simulink model "DemoPromo"  (R2025b)
settings: Solver=VariableStepAuto  StartTime=0.0  StopTime=10.0  RelTol=1e-3
settings Model: Creator=Edward  LastModifiedBy=Edward

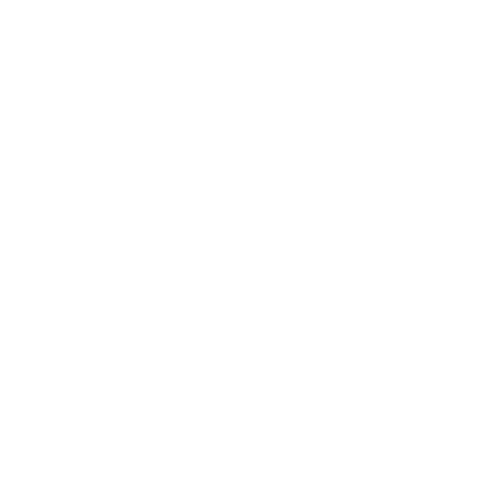
[thumbnail: Simulink's stored preview of the top-level diagram]
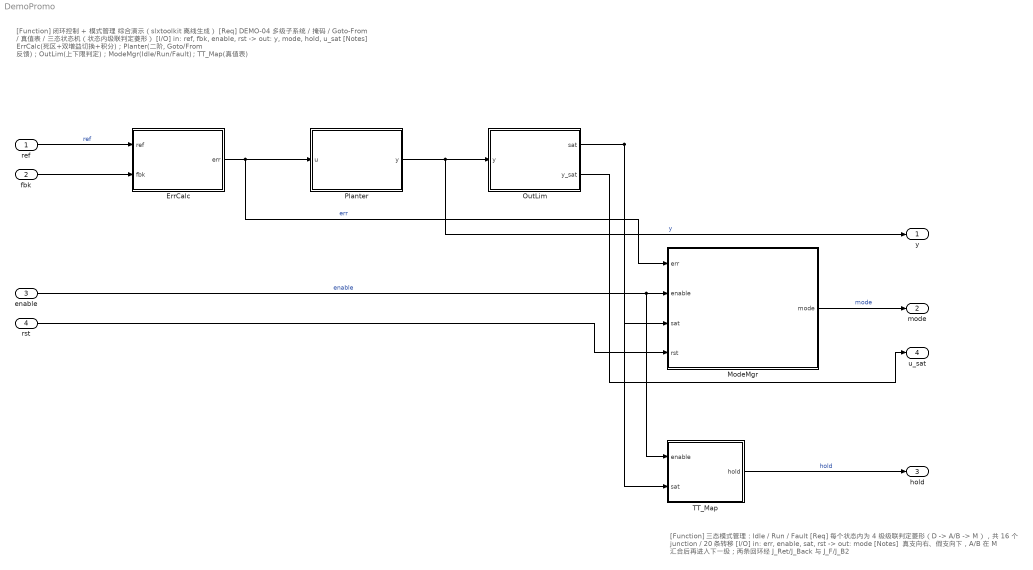
== system DemoPromo ==
  note: [Function] 闭环控制 + 模式管理 综合演示（slxtoolkit 离线生成）
      | [Req] DEMO-04 多级子系统 / 掩码 / Goto-From / 真值表 / 三态状态机（状态内级联判定菱形）
      | [I/O] in: ref, fbk, enable, rst -> out: y, mode, hold, u_sat
      | [Notes] ErrCalc(死区+双增益切换+积分)；Planter(二阶, Goto/From 反馈)；OutLim(上下限判定)；ModeMgr(Idle/Run/Fault)；TT_Map(真值表)
  note: [Function] 三态模式管理：Idle / Run / Fault
      | [Req] 每个状态内为 4 级级联判定菱形（D -> A/B -> M），共 16 个 junction / 20 条转移
      | [I/O] in: err, enable, sat, rst -> out: mode
      | [Notes] 真支向右、假支向下，A/B 在 M 汇合后再进入下一级；两条回环经 J_Ret/J_Back 与 J_F/J_B2
  ref : Inport  OutDataTypeStr=single  PortDimensions=1
  fbk : Inport  OutDataTypeStr=single  PortDimensions=1  Port=2
  enable : Inport  OutDataTypeStr=boolean  PortDimensions=1  Port=3
  rst : Inport  OutDataTypeStr=boolean  PortDimensions=1  Port=4
  ErrCalc : Subsystem  mask(PI Error Calc){Kp=1.5, Kp2=3.0, Ki=0.25}
      mask prompts: Kp "比例增益 Kp"; Kp2 "大误差增益 Kp2"; Ki "积分增益 Ki"
      mask help: 比例 / 积分误差计算（含死区与大误差增益切换），Kp / Kp2 / Ki 由掩码参数给定
      mask DialogControl G_Gain Prompt: PI 增益
      mask DialogControl T_Info Prompt: 仅标定用，运行期不可调
      mask Display: disp('PI error: deadband -> Kp/Kp2 boost -> + Ki integral')
  ModeMgr : Stateflow chart  TreatAsAtomicUnit=on
  OutLim : Subsystem
  Planter : Subsystem
  TT_Map : Truth Table  TreatAsAtomicUnit=on
  y : Outport  OutDataTypeStr=single  PortDimensions=1
  mode : Outport  OutDataTypeStr=uint8  PortDimensions=1  Port=2
  hold : Outport  OutDataTypeStr=boolean  PortDimensions=1  Port=3
  u_sat : Outport  OutDataTypeStr=single  PortDimensions=1  Port=4
  wires:
  ref/1 -> ErrCalc/1(ref)  "ref"
  fbk/1 -> ErrCalc/2(fbk)
  ErrCalc/1(err) -> Planter/1(u), ModeMgr/1(err)  "err"
  Planter/1(y) -> OutLim/1(y), y/1  "y"
  OutLim/1(sat) -> ModeMgr/3(sat), TT_Map/2(sat)
  OutLim/2(y_sat) -> u_sat/1
  enable/1 -> ModeMgr/2(enable), TT_Map/1(enable)  "enable"
  rst/1 -> ModeMgr/4(rst)
  ModeMgr/1(mode) -> mode/1  "mode"
  TT_Map/1(hold) -> hold/1  "hold"

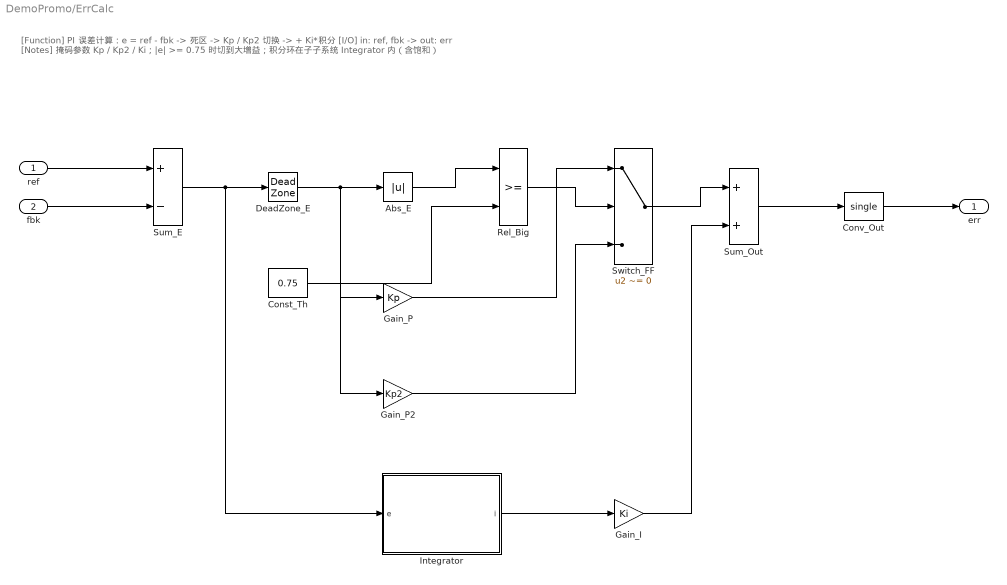
== system DemoPromo/ErrCalc ==
  note: [Function] PI 误差计算：e = ref - fbk -> 死区 -> Kp / Kp2 切换 -> + Ki*积分
      | [I/O] in: ref, fbk -> out: err
      | [Notes] 掩码参数 Kp / Kp2 / Ki；|e| >= 0.75 时切到大增益；积分环在子子系统 Integrator 内（含饱和）
  ref : Inport  OutDataTypeStr=single  PortDimensions=1
  fbk : Inport  OutDataTypeStr=single  PortDimensions=1  Port=2
  Abs_E : Abs
  Const_Th : Constant  Value=0.75  OutDataTypeStr=single  SampleTime=-1
  Conv_Out : DataTypeConversion  OutDataTypeStr=single
  DeadZone_E : DeadZone  LowerValue=-0.0625  UpperValue=0.0625
  Gain_I : Gain  Gain=Ki  OutDataTypeStr=single
  Gain_P : Gain  Gain=Kp  OutDataTypeStr=single
  Gain_P2 : Gain  Gain=Kp2  OutDataTypeStr=single
  Integrator : Subsystem
  Rel_Big : RelationalOperator
  Sum_E : Sum  Inputs=+-
  Sum_Out : Sum
  Switch_FF : Switch  Criteria=u2 ~= 0
  err : Outport  OutDataTypeStr=single  PortDimensions=1
  wires:
  ref/1 -> Sum_E/1
  fbk/1 -> Sum_E/2
  Sum_E/1 -> DeadZone_E/1, Integrator/1(e)
  DeadZone_E/1 -> Abs_E/1, Gain_P/1, Gain_P2/1
  Abs_E/1 -> Rel_Big/1
  Const_Th/1 -> Rel_Big/2
  Gain_P/1 -> Switch_FF/1
  Rel_Big/1 -> Switch_FF/2
  Gain_P2/1 -> Switch_FF/3
  Switch_FF/1 -> Sum_Out/1
  Integrator/1(i) -> Gain_I/1
  Gain_I/1 -> Sum_Out/2
  Sum_Out/1 -> Conv_Out/1
  Conv_Out/1 -> err/1

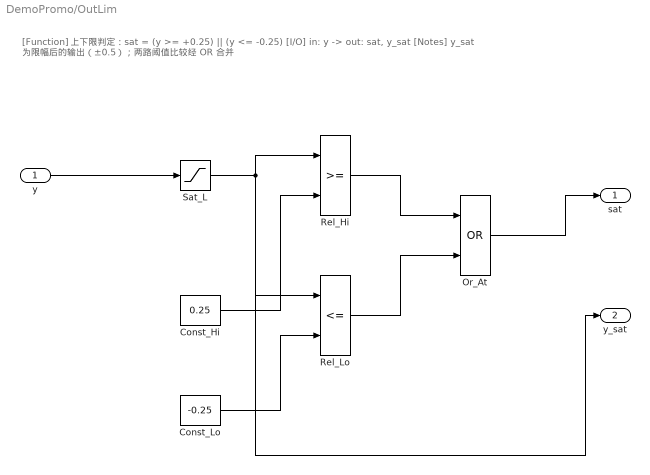
== system DemoPromo/OutLim ==
  note: [Function] 上下限判定：sat = (y >= +0.25) || (y <= -0.25)
      | [I/O] in: y -> out: sat, y_sat
      | [Notes] y_sat 为限幅后的输出（±0.5）；两路阈值比较经 OR 合并
  y : Inport  OutDataTypeStr=single  PortDimensions=1
  Const_Hi : Constant  Value=0.25  OutDataTypeStr=single  SampleTime=-1
  Const_Lo : Constant  Value=-0.25  OutDataTypeStr=single  SampleTime=-1
  Or_At : Logic  Operator=OR
  Rel_Hi : RelationalOperator
  Rel_Lo : RelationalOperator  Operator=<=
  Sat_L : Saturate
  sat : Outport  OutDataTypeStr=boolean  PortDimensions=1
  y_sat : Outport  OutDataTypeStr=single  PortDimensions=1  Port=2
  wires:
  y/1 -> Sat_L/1
  Sat_L/1 -> Rel_Hi/1, Rel_Lo/1, y_sat/1
  Const_Hi/1 -> Rel_Hi/2
  Const_Lo/1 -> Rel_Lo/2
  Rel_Hi/1 -> Or_At/1
  Rel_Lo/1 -> Or_At/2
  Or_At/1 -> sat/1

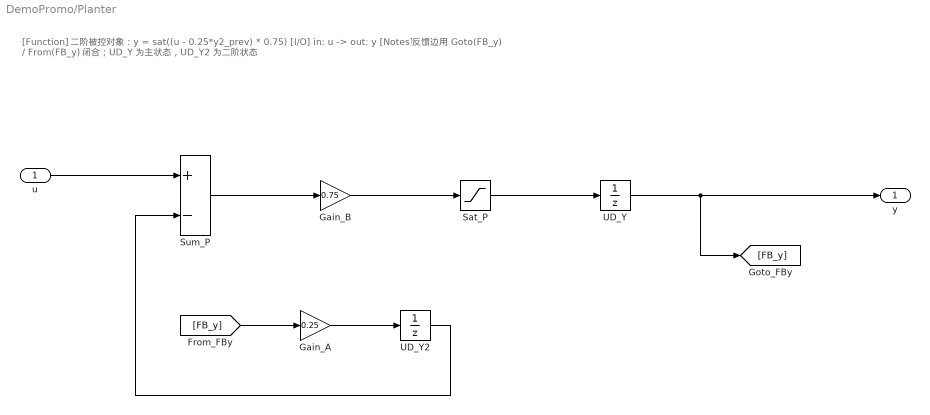
== system DemoPromo/Planter ==
  note: [Function] 二阶被控对象：y = sat((u - 0.25*y2_prev) * 0.75)
      | [I/O] in: u -> out: y
      | [Notes] 反馈边用 Goto(FB_y) / From(FB_y) 闭合；UD_Y 为主状态，UD_Y2 为二阶状态
  u : Inport  OutDataTypeStr=single  PortDimensions=1
  Gain_A : Gain  Gain=0.25  OutDataTypeStr=single
  Gain_B : Gain  Gain=0.75  OutDataTypeStr=single
  Sat_P : Saturate  UpperLimit=1.0  LowerLimit=-1.0
  Sum_P : Sum  Inputs=+-
  UD_Y : UnitDelay  SampleTime=-1
  UD_Y2 : UnitDelay  SampleTime=-1
  y : Outport  OutDataTypeStr=single  PortDimensions=1
  wires:
  u/1 -> Sum_P/1
  Sum_P/1 -> Gain_B/1
  Gain_B/1 -> Sat_P/1
  Sat_P/1 -> UD_Y/1
  UD_Y/1 -> y/1, [FB_y]
  [FB_y] -> Gain_A/1
  Gain_A/1 -> UD_Y2/1
  UD_Y2/1 -> Sum_P/2

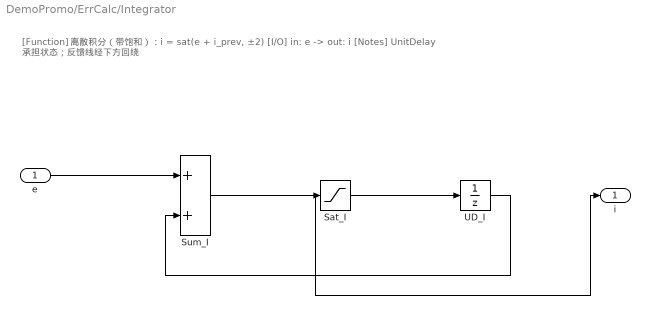
== system DemoPromo/ErrCalc/Integrator ==
  note: [Function] 离散积分（带饱和）：i = sat(e + i_prev, ±2)
      | [I/O] in: e -> out: i
      | [Notes] UnitDelay 承担状态；反馈线经下方回绕
  e : Inport  OutDataTypeStr=single  PortDimensions=1
  Sat_I : Saturate  UpperLimit=2.0  LowerLimit=-2.0
  Sum_I : Sum
  UD_I : UnitDelay  SampleTime=-1
  i : Outport  OutDataTypeStr=single  PortDimensions=1
  wires:
  e/1 -> Sum_I/1
  Sum_I/1 -> Sat_I/1, i/1
  Sat_I/1 -> UD_I/1
  UD_I/1 -> Sum_I/2

== stateflow chart DemoPromo/ModeMgr ==
  state Idle
    en: mode = uint8(0);
    (default) -> (junction 22)
    (junction 22) -> (junction 23) [order 1] : [err < 0.10]
    (junction 22) -> (junction 24) [order 2]
    (junction 23) -> (junction 25)
    (junction 24) -> (junction 25)
    (junction 25) -> (junction 26)
    (junction 26) -> (junction 27) [order 1] : [err < 0.20]
    (junction 26) -> (junction 28) [order 2]
    (junction 27) -> (junction 29)
    (junction 28) -> (junction 29)
    (junction 29) -> (junction 30)
    (junction 30) -> (junction 31) [order 1] : [err < 0.35]
    (junction 30) -> (junction 32) [order 2]
    (junction 31) -> (junction 33)
    (junction 32) -> (junction 33)
    (junction 33) -> (junction 34)
    (junction 34) -> (junction 35) [order 1] : [err < 0.50]
    (junction 34) -> (junction 36) [order 2]
    (junction 35) -> (junction 37)
    (junction 36) -> (junction 37)
  state Run
    en: mode = uint8(1);
    (default) -> (junction 58)
    (junction 58) -> (junction 59) [order 1] : [err < 0.60]
    (junction 58) -> (junction 60) [order 2]
    (junction 59) -> (junction 61)
    (junction 60) -> (junction 61)
    (junction 61) -> (junction 62)
    (junction 62) -> (junction 63) [order 1] : [err < 0.70]
    (junction 62) -> (junction 64) [order 2]
    (junction 63) -> (junction 65)
    (junction 64) -> (junction 65)
    (junction 65) -> (junction 66)
    (junction 66) -> (junction 67) [order 1] : [err < 0.80]
    (junction 66) -> (junction 68) [order 2]
    (junction 67) -> (junction 69)
    (junction 68) -> (junction 69)
    (junction 69) -> (junction 70)
    (junction 70) -> (junction 71) [order 1] : [err < 0.90]
    (junction 70) -> (junction 72) [order 2]
    (junction 71) -> (junction 73)
    (junction 72) -> (junction 73)
  state Fault
    en: mode = uint8(2);
    (default) -> (junction 94)
    (junction 94) -> (junction 95) [order 1] : [err < 0]
    (junction 94) -> (junction 96) [order 2]
    (junction 95) -> (junction 97)
    (junction 96) -> (junction 97)
  (default) -> Idle
  Idle -> Run : [enable]
  Run -> Fault [order 2] : [sat]
  Fault -> (junction 11) : [rst]{mode = uint8(0);}
  (junction 10) -> Idle
  Run -> (junction 9) [order 1] : [enable == false]
  (junction 9) -> (junction 10)
  (junction 12) -> (junction 10)
  (junction 11) -> (junction 12)
  data: err input single size=1; enable input boolean size=1; sat input boolean size=1; rst input boolean size=1; mode output uint8 size=1

== matlab function DemoPromo/TT_Map ==
  data: enable input boolean; sat input boolean; hold output boolean
function hold = fcn(enable, sat)

aVarTruthTableCondition_1 = false;
aVarTruthTableCondition_2 = false;


% 使能

aVarTruthTableCondition_1 = logical(enable);

% 饱和

aVarTruthTableCondition_2 = logical(sat);

if (aVarTruthTableCondition_1 && aVarTruthTableCondition_2)
    aFcnTruthTableAction_1();
elseif (aVarTruthTableCondition_1 && ~aVarTruthTableCondition_2)
    aFcnTruthTableAction_2();
else % Default
    aFcnTruthTableAction_2();
end

function aFcnTruthTableAction_1()

    % 保持

    hold = true;

function aFcnTruthTableAction_2()

    % 释放

    hold = false;
